simulink model "Inverted_Pendulum_Model"  (R2024b)
settings: Solver=VariableStepAuto  StartTime=0.0  StopTime=10.0  MaxStep=.001  RelTol=1e-3
model workspace (MAT data in the model file):
  M = 0.5
  N = 100
  b = 0.1
  g = 9.81
  l = 0.3
  m = 0.2
undefined symbols (not defined in the file): L
settings Model: Creator=Mohamed  LastModifiedBy=Mohamed

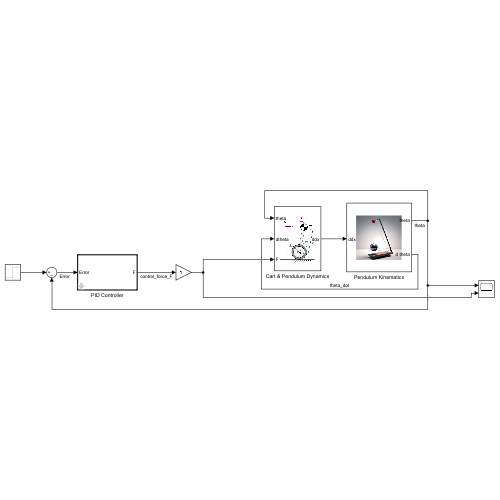
[thumbnail: Simulink's stored preview of the top-level diagram]
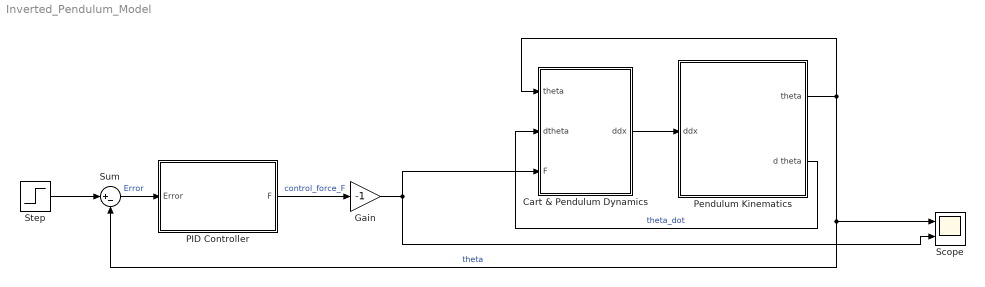
== system Inverted_Pendulum_Model ==
  Cart & Pendulum Dynamics : Subsystem
      mask Display: image('images.png', [0,0,0,0,90,70]);
  Gain : Gain  Gain=-1
  PID Controller : Subsystem  TreatAsAtomicUnit=on  mask{kp=40, ki=5, Kd=12, N=100}
  Pendulum Kinematics : Subsystem
      mask Display: image('images.jpg', [0,0,0,0,70,70]);
  Scope : Scope  NumInputPorts=2
  Step : Step  After=.0  SampleTime=0
  Sum : Sum  Inputs=|+-
  wires:
  Cart & Pendulum Dynamics/1(ddx) -> Pendulum Kinematics/1(ddx)
  Pendulum Kinematics/1(theta) -> Scope/1, Sum/2, Cart & Pendulum Dynamics/1(theta)  "theta"
  Pendulum Kinematics/2(d theta) -> Cart & Pendulum Dynamics/2(dtheta)  "theta_dot"
  Step/1 -> Sum/1
  Sum/1 -> PID Controller/1(Error)  "Error"
  PID Controller/1(F) -> Gain/1  "control_force_F"
  Gain/1 -> Cart & Pendulum Dynamics/3(F), Scope/2

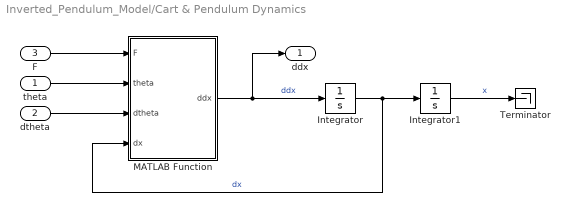
== system Inverted_Pendulum_Model/Cart & Pendulum Dynamics ==
  theta : Inport
  dtheta : Inport  Port=2
  F : Inport  Port=3
  Integrator : Integrator
  Integrator1 : Integrator
  MATLAB Function : MATLAB Function  TreatAsAtomicUnit=on
  Terminator : Terminator
  ddx : Outport
  wires:
  theta/1 -> MATLAB Function/2(theta)
  MATLAB Function/1(ddx) -> ddx/1, Integrator/1  "ddx"
  dtheta/1 -> MATLAB Function/3(dtheta)
  Integrator1/1 -> Terminator/1  "x"
  F/1 -> MATLAB Function/1(F)
  Integrator/1 -> MATLAB Function/4(dx), Integrator1/1  "dx"

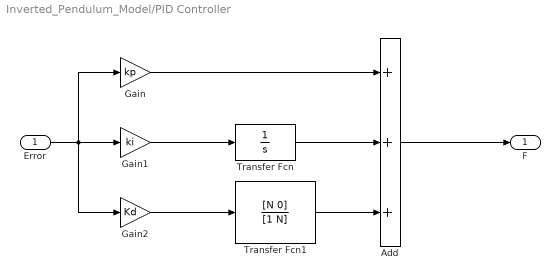
== system Inverted_Pendulum_Model/PID Controller ==
  Error : Inport
  Add : Sum  Inputs=+++
  Gain : Gain  Gain=kp
  Gain1 : Gain  Gain=ki
  Gain2 : Gain  Gain=Kd
  Transfer Fcn : TransferFcn  Denominator=[1 0]
  Transfer Fcn1 : TransferFcn  Numerator=[N 0]  Denominator=[1 N]
  F : Outport
  wires:
  Gain/1 -> Add/1
  Transfer Fcn/1 -> Add/2
  Gain1/1 -> Transfer Fcn/1
  Gain2/1 -> Transfer Fcn1/1
  Transfer Fcn1/1 -> Add/3
  Add/1 -> F/1
  Error/1 -> Gain2/1, Gain/1, Gain1/1

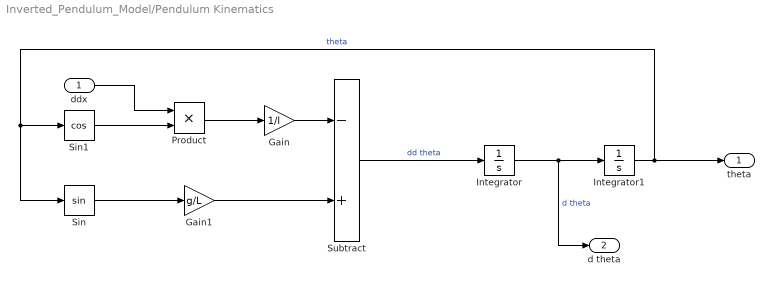
== system Inverted_Pendulum_Model/Pendulum Kinematics ==
  ddx : Inport
  Gain : Gain  Gain=1/l
  Gain1 : Gain  Gain=g/L
  Integrator : Integrator
  Integrator1 : Integrator  InitialCondition=0.087
  Product : Product
  Sin : Trigonometry
  Sin1 : Trigonometry  Operator=cos
  Subtract : Sum  Inputs=-+
  theta : Outport
  d theta : Outport  Port=2
  wires:
  Sin/1 -> Gain1/1
  Subtract/1 -> Integrator/1  "dd theta"
  Product/1 -> Gain/1
  Integrator1/1 -> theta/1, Sin/1, Sin1/1  "theta"
  Gain/1 -> Subtract/1
  Integrator/1 -> d theta/1, Integrator1/1  "d theta"
  ddx/1 -> Product/1
  Sin1/1 -> Product/2
  Gain1/1 -> Subtract/2

== matlab function Inverted_Pendulum_Model/Cart & Pendulum Dynamics/MATLAB Function ==
  data: F input; theta input; dtheta input; dx input; ddx output; g parameter; M parameter; l parameter; m parameter; b parameter
function ddx = fcn(F,theta,dtheta,dx,g, M, l, m, b)

ddx = 1/(M + m*(sin(theta))^2)*(F + m*l*dtheta^2*sin(theta) -b*dx -m*g*cos(theta)*sin(theta));
end
